simulink library "tip_assist_lib_support"  (Simulink 9.0)
settings: Solver=VariableStepAuto  StartTime=0.0  StopTime=10.0  RelTol=1e-3
undefined symbols (not defined in the file): g, timestep, TipAssistAdvEcmError_t, TipAssistCpmTipOffMode_t, TipAssistLiveWeighStatus_t, TipAssistPayloadType_t, TipAssistSecPfwStatus_t, TipAssistUnsecPfwStatus_t, toa_appNumber, toa_expectedBucketAngNoise, toa_imu_lpf_cutoff_hz, toa_imuBasicOrient, toa_liftBoreDia, toa_liftRodDia, toa_liveLpfCutoffHz, toa_liveSpillRateLpfCutoffHz, toa_mcGroundCombBucketAng, toa_mcGroundCombLiftNormAng, toa_mcGroundLiftNormAng, toa_noSlidingAngle, toa_payload_target_ov_val, toa_payloadTargetMin, toa_pfwLpfCutoffHz, toa_pfwResetLpfCutoffHz, toa_pfwResetStatsBound, toa_pfwResetStatsConf, toa_pfwTiltNormRackThresh, toa_pfwTravelExtentLower, toa_pfwTravelExtentUpper, toa_ratedPayload, toa_reposeMarginAng, toa_sendCpmLiveLpfCutoffHz, toa_sendToCpmMinPrecision, toa_tiltBoreDia, toa_tiltNumCyl, toa_tiltRodDia, toa_toolBcAngle, toa_toolBcLength
libraries: lib_CATutils_Utilities_ApplyName_v2 x113, simulink x18, tip_assist_lib x14, lib_CATutils_Filters_1Pole_LowPass x6, simulink_extras x5, lib_CATutils_Override x3, lib_CATutils_Hysteresis_Latch x3, lib_CATutils_Timer_Countdown x3, tip_assist_lib_support x2
(part 3 of 4)

== system tip_assist_lib_support/Tip-Off Assist Support Lib/Tip-Off Assist Payload/Pseudo-Frictionless Weigh/Notch filter ==
  in : Inport
  reset : Inport  Port=2
  NotchFilter : Subsystem  mask{mskCutoffFreqRadPerSec=5.0}
      mask prompts: mskCutoffFreqRadPerSec "Cutoff Frequency (rad/s)"
      settings: AttributesFormatString=cf: %<mskCutoffFreqRadPerSec>
  NotchFilter1 : Subsystem  mask{mskCutoffFreqRadPerSec=7.5}
      mask prompts: mskCutoffFreqRadPerSec "Cutoff Frequency (rad/s)"
      settings: AttributesFormatString=cf: %<mskCutoffFreqRadPerSec>
  NotchFilter2 : Subsystem  mask{mskCutoffFreqRadPerSec=12.0}
      mask prompts: mskCutoffFreqRadPerSec "Cutoff Frequency (rad/s)"
      settings: AttributesFormatString=cf: %<mskCutoffFreqRadPerSec>
  out : Outport
  wires:
  NotchFilter/1(filtered) -> NotchFilter1/1(raw)
  NotchFilter1/1(filtered) -> NotchFilter2/1(raw)
  reset/1 -> NotchFilter2/2(reset), NotchFilter1/2(reset), NotchFilter/2(reset)
  in/1 -> NotchFilter/1(raw)
  NotchFilter2/1(filtered) -> out/1

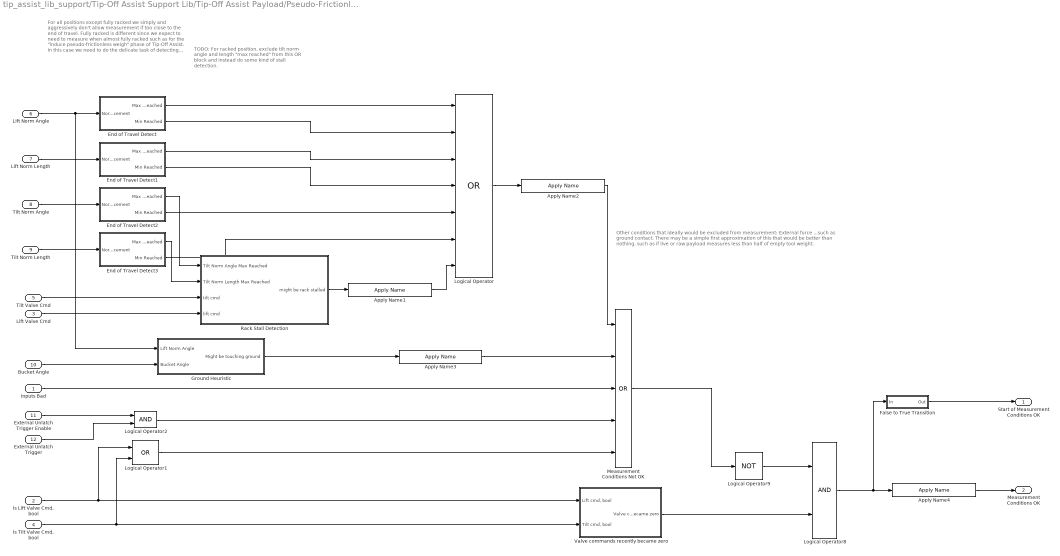
== system tip_assist_lib_support/Tip-Off Assist Support Lib/Tip-Off Assist Payload/Pseudo-Frictionless Weigh/Pseudo-Frictionless Weigh Common Measurement Conditions ==
  note: Other conditions that ideally would be excluded from measurement:
      |
      | External force
      | ...such as ground contact.  There may be a simple first approximation of this that would be better than nothing, such as if live or raw payload measures less than half of empty tool weight.
  note: TODO: For racked position, exclude tilt norm angle and length "max reached" from this OR block and instead do some kind of stall detection.
  note: For all positions except fully racked we simply and aggressively don't allow measurement if too close to the end of travel.
      |
      | Fully racked is different since we expect to need to measure when almost fully racked such as for the "induce pseudo-frictionless weigh" phase of Tip-Off Assist.  In this case we need to do the delicate task of detecting when we are definitely off the rack stops and not hitting the end of tilt cylinder stroke, even if we are close to either.
  Inputs Bad : Inport
  "Is Lift Valve Cmd, bool" : Inport  Port=2
  Lift Valve Cmd : Inport  Port=3
  "Is Tilt Valve Cmd, bool" : Inport  Port=4
  Tilt Valve Cmd : Inport  Port=5
  "Lift Norm Angle " : Inport  Port=6
  Lift Norm Length : Inport  Port=7
  Tilt Norm Angle : Inport  Port=8
  Tilt Norm Length : Inport  Port=9
  Bucket Angle : Inport  Port=10
  External Unlatch Trigger Enable : Inport  Port=11
  External Unlatch Trigger : Inport  Port=12
  Apply Name1 : lib_CATutils_Utilities_ApplyName_v2/Apply Name  sigLabel='toa_pfwMcMaybeRackStall'  enTst=true
  Apply Name2 : lib_CATutils_Utilities_ApplyName_v2/Apply Name  sigLabel='toa_pfwMcMaybeStalled'  enTst=true
  Apply Name3 : lib_CATutils_Utilities_ApplyName_v2/Apply Name  sigLabel='toa_pfwMcMaybeGrounded'  enTst=true
  Apply Name4 : lib_CATutils_Utilities_ApplyName_v2/Apply Name  sigLabel='toa_pfwMcOk'  enTst=true
  End of Travel Detect : Subsystem
  End of Travel Detect1 : Subsystem
  End of Travel Detect2 : Subsystem
  End of Travel Detect3 : Subsystem
  False to True Transition : Subsystem
  Ground Heuristic : Subsystem
  Logical Operator : Logic  Operator=OR  Inputs=7  AllPortsSameDT=off  OutDataTypeStr=boolean
  Logical Operator2 : Logic  AllPortsSameDT=off  OutDataTypeStr=boolean
  Logical Operator1 : Logic  Operator=OR
  Logical Operator8 : Logic
  Logical Operator9 : Logic  Operator=NOT
  Measurement Conditions Not OK : Logic  Operator=OR  Inputs=5  AllPortsSameDT=off  OutDataTypeStr=boolean
  Rack Stall Detection : Subsystem
  Valve commands recently became zero : Subsystem
  Start of Measurement Conditions OK : Outport
  Measurement Conditions OK : Outport  Port=2
  wires:
  False to True Transition/1(Out) -> Start of Measurement Conditions OK/1
  Logical Operator8/1 -> Apply Name4/1, False to True Transition/1(In)
  Inputs Bad/1 -> Measurement Conditions Not OK/3
  Logical Operator9/1 -> Logical Operator8/1
  "Is Lift Valve Cmd, bool"/1 -> Logical Operator1/1, Valve commands recently became zero/1("Lift cmd, bool")
  "Is Tilt Valve Cmd, bool"/1 -> Logical Operator1/2, Valve commands recently became zero/2("Tilt cmd, bool")
  Valve commands recently became zero/1(Valve cmd recently became zero) -> Logical Operator8/2
  Logical Operator/1 -> Apply Name2/1
  Logical Operator1/1 -> Measurement Conditions Not OK/5
  Measurement Conditions Not OK/1 -> Logical Operator9/1
  "Lift Norm Angle "/1 -> Ground Heuristic/1(Lift Norm Angle), End of Travel Detect/1(Normalized Displacement)
  Lift Norm Length/1 -> End of Travel Detect1/1(Normalized Displacement)
  Tilt Norm Angle/1 -> End of Travel Detect2/1(Normalized Displacement)
  End of Travel Detect/2(Min Reached) -> Logical Operator/2
  End of Travel Detect/1(Max Reached) -> Logical Operator/1
  End of Travel Detect1/2(Min Reached) -> Logical Operator/4
  End of Travel Detect1/1(Max Reached) -> Logical Operator/3
  End of Travel Detect2/2(Min Reached) -> Logical Operator/5
  Tilt Norm Length/1 -> End of Travel Detect3/1(Normalized Displacement)
  End of Travel Detect3/2(Min Reached) -> Logical Operator/6
  External Unlatch Trigger/1 -> Logical Operator2/2
  External Unlatch Trigger Enable/1 -> Logical Operator2/1
  Logical Operator2/1 -> Measurement Conditions Not OK/4
  Bucket Angle/1 -> Ground Heuristic/2(Bucket Angle)
  Ground Heuristic/1(Might be touching ground) -> Apply Name3/1
  End of Travel Detect2/1(Max Reached) -> Rack Stall Detection/1(Tilt Norm Angle Max Reached)
  End of Travel Detect3/1(Max Reached) -> Rack Stall Detection/2(Tilt Norm Length Max Reached)
  Tilt Valve Cmd/1 -> Rack Stall Detection/3(tilt cmd)
  Lift Valve Cmd/1 -> Rack Stall Detection/4(lift cmd)
  Rack Stall Detection/1(might be rack stalled) -> Apply Name1/1
  Apply Name4/1 -> Measurement Conditions OK/1
  Apply Name1/1 -> Logical Operator/7
  Apply Name2/1 -> Measurement Conditions Not OK/1
  Apply Name3/1 -> Measurement Conditions Not OK/2

== system tip_assist_lib_support/Tip-Off Assist Support Lib/Tip-Off Assist Payload/Pseudo-Frictionless Weigh/Racked ==
  note: Racking maxes out norm angle or length depending on on lift position. So if one of those is close to 1 we will assume we're racked.
  Tilt Norm Angle : Inport
  Tilt Norm Length : Inport  Port=2
  Add1 : Sum  Inputs=-+
  Data Type Conversion : DataTypeConversion  OutDataTypeStr=boolean
  Latched Point Hysteresis : lib_CATutils_Hysteresis_Latch/Latched Point Hysteresis  extBreakPoints=on  Min_Break_Point=-0.5  Max_Break_Point=0.5  extValues=off  Lo_Value=0  Hi_Value=1  Out_Mode=unused and invalid  Out_DataType=[]  Out_Scaling=[]  OutDataTypeStr=int8
  MinMax : MinMax  Function=max  Inputs=2
  "expected bucket angle noise amplitude, deg" : Constant  Value=toa_expectedBucketAngNoise  OutDataTypeStr=single  SampleTime=-1
  guessed typical ratio of tilt norm angle to bucket angle : Gain  Gain=0.0075
  min tilt norm angle to be considered racked : Constant  Value=toa_pfwTiltNormRackThresh  OutDataTypeStr=single  SampleTime=-1
  "Assume racked, bool" : Outport
  wires:
  Tilt Norm Angle/1 -> MinMax/1
  Data Type Conversion/1 -> "Assume racked, bool"/1
  "expected bucket angle noise amplitude, deg"/1 -> guessed typical ratio of tilt norm angle to bucket angle/1
  Add1/1 -> Latched Point Hysteresis/2
  Latched Point Hysteresis/1 -> Data Type Conversion/1
  min tilt norm angle to be considered racked/1 -> Add1/2, Latched Point Hysteresis/3
  guessed typical ratio of tilt norm angle to bucket angle/1 -> Add1/1
  Tilt Norm Length/1 -> MinMax/2
  MinMax/1 -> Latched Point Hysteresis/1

== system tip_assist_lib_support/Tip-Off Assist Support Lib/Tip-Off Assist Payload/Pseudo-Frictionless Weigh/Secure Latched Payload (resets to NaN) ==
  set : Inport
  reset : Inport  Port=2
  signal : Inport  Port=3
  Unit Delay : UnitDelay  InitialCondition=mskInitialOut  SampleTime=-1
      settings: AttributesFormatString=IC: %<X0>
  false : Constant  Value=mskInitialOut  OutDataTypeStr=Inherit: Inherit via back propagation  SampleTime=-1
  resetSwitch : Switch  Criteria=u2 ~= 0  InputSameDT=on
      settings: AttributesFormatString=%<Criteria>
  setSwitch : Switch  Criteria=u2 ~= 0  InputSameDT=on
      settings: AttributesFormatString=%<Criteria>
  out : Outport
  wires:
  reset/1 -> resetSwitch/2
  setSwitch/1 -> resetSwitch/3
  set/1 -> setSwitch/2
  false/1 -> resetSwitch/1
  signal/1 -> setSwitch/1
  resetSwitch/1 -> out/1, Unit Delay/1
  Unit Delay/1 -> setSwitch/3

== system tip_assist_lib_support/Tip-Off Assist Support Lib/Tip-Off Assist Payload/Pseudo-Frictionless Weigh/Secure Latched Standard Deviation (resets to inf) ==
  set : Inport
  reset : Inport  Port=2
  signal : Inport  Port=3
  Unit Delay : UnitDelay  InitialCondition=mskInitialOut  SampleTime=-1
      settings: AttributesFormatString=IC: %<X0>
  false : Constant  Value=mskInitialOut  OutDataTypeStr=Inherit: Inherit via back propagation  SampleTime=-1
  resetSwitch : Switch  Criteria=u2 ~= 0  InputSameDT=on
      settings: AttributesFormatString=%<Criteria>
  setSwitch : Switch  Criteria=u2 ~= 0  InputSameDT=on
      settings: AttributesFormatString=%<Criteria>
  out : Outport
  wires:
  Unit Delay/1 -> setSwitch/3
  resetSwitch/1 -> Unit Delay/1, out/1
  signal/1 -> setSwitch/1
  false/1 -> resetSwitch/1
  set/1 -> setSwitch/2
  setSwitch/1 -> resetSwitch/3
  reset/1 -> resetSwitch/2

== system tip_assist_lib_support/Tip-Off Assist Support Lib/Tip-Off Assist Payload/Pseudo-Frictionless Weigh/Secure Payload Latch State ==
  set : Inport
  reset : Inport  Port=2
  Unit Delay : UnitDelay  InitialCondition=mskInitialOut  SampleTime=-1
      settings: AttributesFormatString=IC: %<X0>
  false : Constant  Value=0  OutDataTypeStr=boolean
  resetSwitch : Switch  Criteria=u2 ~= 0  InputSameDT=on
      settings: AttributesFormatString=%<Criteria>
  setSwitch : Switch  Criteria=u2 ~= 0  InputSameDT=on
      settings: AttributesFormatString=%<Criteria>
  true : Constant  OutDataTypeStr=boolean
  out : Outport
  wires:
  Unit Delay/1 -> setSwitch/3
  resetSwitch/1 -> Unit Delay/1, out/1
  true/1 -> setSwitch/1
  false/1 -> resetSwitch/1
  set/1 -> setSwitch/2
  setSwitch/1 -> resetSwitch/3
  reset/1 -> resetSwitch/2

== system tip_assist_lib_support/Tip-Off Assist Support Lib/Tip-Off Assist Payload/Pseudo-Frictionless Weigh/Secure Payload Unlatch Logic ==
  note: When external unlatch is disabled, the non-command unlatch signals become relevant if slope is used. The noise in the slope would need to be accounted for somewhere to prevent accidental unlatching.
  Lift Cmd : Inport
  Tilt Cmd : Inport  Port=2
  External Unlatch Trigger Enable : Inport  Port=3
  External Unlatch Trigger : Inport  Port=4
  Unsecure Transition Unlatch Trigger : Inport  Port=5
  Apply Name1 : lib_CATutils_Utilities_ApplyName_v2/Apply Name  sigLabel='toa_pfwLatchInvalidate'  enTst=true
  Logical Operator2 : Logic  Operator=OR  AllPortsSameDT=off  OutDataTypeStr=boolean
  Logical Operator3 : Logic  Operator=OR  AllPortsSameDT=off  OutDataTypeStr=boolean
  Switch : Switch  Criteria=u2 ~= 0
  Unlatch Out : Outport
  wires:
  Switch/1 -> Apply Name1/1
  External Unlatch Trigger/1 -> Logical Operator3/1
  External Unlatch Trigger Enable/1 -> Switch/2
  Lift Cmd/1 -> Logical Operator2/1
  Tilt Cmd/1 -> Logical Operator2/2
  Logical Operator2/1 -> Switch/3
  Unsecure Transition Unlatch Trigger/1 -> Logical Operator3/2
  Logical Operator3/1 -> Switch/1
  Apply Name1/1 -> Unlatch Out/1

== system tip_assist_lib_support/Tip-Off Assist Support Lib/Tip-Off Assist Payload/Pseudo-Frictionless Weigh/Sliding ==
  "Bucket Angle, deg" : Inport
  Add1 : Sum
  Data Type Conversion : DataTypeConversion  OutDataTypeStr=boolean
  Latched Point Hysteresis : lib_CATutils_Hysteresis_Latch/Latched Point Hysteresis  extBreakPoints=on  Min_Break_Point=-0.5  Max_Break_Point=0.5  extValues=off  Lo_Value=0  Hi_Value=1  Out_Mode=unused and invalid  Out_DataType=[]  Out_Scaling=[]  OutDataTypeStr=int8
  "expected bucket angle noise amplitude, deg" : Constant  Value=toa_expectedBucketAngNoise  OutDataTypeStr=single  SampleTime=-1
  "sliding threshold, degrees" : Constant  Value=toa_noSlidingAngle  OutDataTypeStr=single  SampleTime=-1
  "Assume no sliding, bool" : Outport
  "Bucket angle of no sliding threshold, deg" : Outport  Port=2
  wires:
  "sliding threshold, degrees"/1 -> "Bucket angle of no sliding threshold, deg"/1, Add1/1, Latched Point Hysteresis/2
  Latched Point Hysteresis/1 -> Data Type Conversion/1
  Add1/1 -> Latched Point Hysteresis/3
  "expected bucket angle noise amplitude, deg"/1 -> Add1/2
  Data Type Conversion/1 -> "Assume no sliding, bool"/1
  "Bucket Angle, deg"/1 -> Latched Point Hysteresis/1

== system tip_assist_lib_support/Tip-Off Assist Support Lib/Tip-Off Assist Payload/Pseudo-Frictionless Weigh/Statistics Estimation1 ==
  note: A good variance to reset the filter to is the variance that corresponds to the distribution whose confidence interval at the prescribed confidence (99.7%) has a half-width (aka bound) that is 75% of the rated payload.
      |
      | This is like saying that we're always 99.7% sure that the true payload is within 75% of rated payload of our raw measurement.
  Signal In : Inport
  Low Pass Filter Cutoff (Hz) : Inport  Port=2
  Reset : Inport  Port=3
  "Rated Payload, t" : Inport  Port=4
  Constant : Constant  Value=toa_pfwResetStatsConf  OutDataTypeStr=single  SampleTime=-1
  Constant1 : Constant  Value=toa_pfwResetStatsBound  OutDataTypeStr=single  SampleTime=-1
  Constant2 : Constant  Value=timestep  SampleTime=timestep
  MATLAB Function : MATLAB Function  TreatAsAtomicUnit=on
  MATLAB Function1 : tip_assist_lib/MATLAB Function
  Math Function : Math  Operator=square  SaturateOnIntegerOverflow=on
  Product : Product
  Two Sided St. Dev. from Bound : MATLAB Function  TreatAsAtomicUnit=on
  stdevEst : Outport
  meanEst : Outport  Port=2
  wires:
  Reset/1 -> MATLAB Function/3(reset)
  MATLAB Function1/1 -> MATLAB Function/2(filterFactor)
  Low Pass Filter Cutoff (Hz)/1 -> MATLAB Function1/2
  Constant2/1 -> MATLAB Function1/1
  MATLAB Function/2(stdevEst) -> stdevEst/1
  MATLAB Function/1(meanEst) -> meanEst/1
  Signal In/1 -> MATLAB Function/4(resetSample), MATLAB Function/1(newSample)
  "Rated Payload, t"/1 -> Product/1
  Constant/1 -> Two Sided St. Dev. from Bound/1(confidence)
  Math Function/1 -> MATLAB Function/5(resetVariance)
  Two Sided St. Dev. from Bound/1(stdev) -> Math Function/1
  Constant1/1 -> Product/2
  Product/1 -> Two Sided St. Dev. from Bound/2(bound)

== system tip_assist_lib_support/Tip-Off Assist Support Lib/Tip-Off Assist Payload/Pseudo-Frictionless Weigh/Statistics Estimation2 ==
  note: A good variance to reset the filter to is the variance that corresponds to the distribution whose confidence interval at the prescribed confidence (99.7%) has a half-width (aka bound) that is 75% of the rated payload.
      |
      | This is like saying that we're always 99.7% sure that the true payload is within 75% of rated payload of our raw measurement.
  Signal In : Inport
  Low Pass Filter Cutoff (Hz) : Inport  Port=2
  Reset : Inport  Port=3
  "Rated Payload, t" : Inport  Port=4
  Constant : Constant  Value=toa_pfwResetStatsConf  OutDataTypeStr=single  SampleTime=-1
  Constant1 : Constant  Value=toa_pfwResetStatsBound  OutDataTypeStr=single  SampleTime=-1
  Constant2 : Constant  Value=timestep  SampleTime=timestep
  MATLAB Function : MATLAB Function  TreatAsAtomicUnit=on
  MATLAB Function1 : tip_assist_lib/MATLAB Function
  Math Function : Math  Operator=square  SaturateOnIntegerOverflow=on
  Product : Product
  Two Sided St. Dev. from Bound : MATLAB Function  TreatAsAtomicUnit=on
  stdevEst : Outport
  meanEst : Outport  Port=2
  wires:
  Product/1 -> Two Sided St. Dev. from Bound/2(bound)
  Constant1/1 -> Product/2
  Two Sided St. Dev. from Bound/1(stdev) -> Math Function/1
  Math Function/1 -> MATLAB Function/5(resetVariance)
  Constant/1 -> Two Sided St. Dev. from Bound/1(confidence)
  "Rated Payload, t"/1 -> Product/1
  Signal In/1 -> MATLAB Function/4(resetSample), MATLAB Function/1(newSample)
  MATLAB Function/1(meanEst) -> meanEst/1
  MATLAB Function/2(stdevEst) -> stdevEst/1
  Constant2/1 -> MATLAB Function1/1
  Low Pass Filter Cutoff (Hz)/1 -> MATLAB Function1/2
  MATLAB Function1/1 -> MATLAB Function/2(filterFactor)
  Reset/1 -> MATLAB Function/3(reset)

== system tip_assist_lib_support/Tip-Off Assist Support Lib/Tip-Off Assist Payload/Pseudo-Frictionless Weigh/Sure dig is over ==
  note: need a set/reset block here so we can only call a dig over if we previously knew a dig was happening
  note: need a timer here so that if dig starts but we never see anything saying its over we call it over a certain amount of time after dig state becomes false
  note: need a block here that looks for a definite dump
  Dig State : Inport
  Ground Speed : Inport  Port=2
  Ground Speed1 : Inport  Port=3
  Tilt Cmd : Inport  Port=4
  Logical Operator : Logic  Operator=OR  AllPortsSameDT=off  OutDataTypeStr=boolean
  Dig Definitely Done event : Outport
  wires:
  Dig State/1 -> ?
  Logical Operator/1 -> Dig Definitely Done event/1

== system tip_assist_lib_support/Tip-Off Assist Support Lib/Tip-Off Assist Payload/Pseudo-Frictionless Weigh/Variance Anti-Noise Filter1 ==
  note: Per Aaron Shatters:
      | This filter was added to PCS (the CPM predecessor) because pump piston pass frequency was aliasing into the signal.  Being kind of like a discrete derivative, the variance calculation is sensitive to high frequency noise.  So this filter was added to prevent the high frequency instances of this noise.  Being a two sample moving average, it is the fastest filter that eliminated the noise.  It was not thoroughly technically examined, but it worked.  It's not clear the extent to which this is necessary here, since Pseudo-Frictionless Weigh works only when the tilt and lift valve command is zero, so the pump should not be hydraulically connected to the cylinder at this time.  The pump is also likely to be at a low stroke, so piston pass ripple amplitude should be low.
  in : Inport
  reset : Inport  Port=2
  MATLAB Function : MATLAB Function  TreatAsAtomicUnit=on
  out : Outport
  wires:
  reset/1 -> MATLAB Function/2(reset)
  in/1 -> MATLAB Function/1(u)
  MATLAB Function/1(y) -> out/1

== system tip_assist_lib_support/Tip-Off Assist Support Lib/Tip-Off Assist Payload/Pseudo-Frictionless Weigh/Variance Anti-Noise Filter2 ==
  note: Per Aaron Shatters:
      | This filter was added to PCS (the CPM predecessor) because pump piston pass frequency was aliasing into the signal.  Being kind of like a discrete derivative, the variance calculation is sensitive to high frequency noise.  So this filter was added to prevent the high frequency instances of this noise.  Being a two sample moving average, it is the fastest filter that eliminated the noise.  It was not thoroughly technically examined, but it worked.  It's not clear the extent to which this is necessary here, since Pseudo-Frictionless Weigh works only when the tilt and lift valve command is zero, so the pump should not be hydraulically connected to the cylinder at this time.  The pump is also likely to be at a low stroke, so piston pass ripple amplitude should be low.
  in : Inport
  reset : Inport  Port=2
  MATLAB Function : MATLAB Function  TreatAsAtomicUnit=on
  out : Outport
  wires:
  MATLAB Function/1(y) -> out/1
  in/1 -> MATLAB Function/1(u)
  reset/1 -> MATLAB Function/2(reset)

== system tip_assist_lib_support/Tip-Off Assist Support Lib/Tip-Off Assist Payload/Pseudo-Frictionless Weigh/Weighing Statistics, No Notch, No Latch ==
  PFW Payload Std. Dev. : Inport
  PFW Payload Mean : Inport  Port=2
  Add : Sum
  Add1 : Sum
  Constant : Constant  Value=0.997
  One Sided Confidence Limit : MATLAB Function  TreatAsAtomicUnit=on
  Subtract : Sum  Inputs=+-
  Subtract1 : Sum  Inputs=+-
  Two Sided Confidence Limit : MATLAB Function  TreatAsAtomicUnit=on
  One Sided Payload Upper Bound : Outport
  One Sided Payload Lower Bound : Outport  Port=2
  One Sided Payload Bound Size : Outport  Port=3
  Two Sided Payload Upper Bound : Outport  Port=4
  Two Sided Payload Lower Bound : Outport  Port=5
  Two Sided Payload Bound Size : Outport  Port=6
  wires:
  PFW Payload Mean/1 -> Subtract1/1, Add1/2, Subtract/1, Add/2
  PFW Payload Std. Dev./1 -> Two Sided Confidence Limit/2(stdev), One Sided Confidence Limit/2(stdev)
  Constant/1 -> One Sided Confidence Limit/1(confidence), Two Sided Confidence Limit/1(confidence)
  One Sided Confidence Limit/1(bound) -> Subtract/2, Add/1, One Sided Payload Bound Size/1
  Add/1 -> One Sided Payload Upper Bound/1
  Subtract/1 -> One Sided Payload Lower Bound/1
  Two Sided Confidence Limit/1(bound) -> Subtract1/2, Add1/1, Two Sided Payload Bound Size/1
  Add1/1 -> Two Sided Payload Upper Bound/1
  Subtract1/1 -> Two Sided Payload Lower Bound/1

== system tip_assist_lib_support/Tip-Off Assist Support Lib/Tip-Off Assist Payload/Pseudo-Frictionless Weigh/Weighing Statistics, Notch, No Latch ==
  PFW Payload Std. Dev. : Inport
  PFW Payload Mean : Inport  Port=2
  Add : Sum
  Add1 : Sum
  Constant : Constant  Value=0.997
  One Sided Confidence Limit : MATLAB Function  TreatAsAtomicUnit=on
  Subtract : Sum  Inputs=+-
  Subtract1 : Sum  Inputs=+-
  Two Sided Confidence Limit : MATLAB Function  TreatAsAtomicUnit=on
  One Sided Payload Upper Bound : Outport
  One Sided Payload Lower Bound : Outport  Port=2
  One Sided Payload Bound Size : Outport  Port=3
  Two Sided Payload Upper Bound : Outport  Port=4
  Two Sided Payload Lower Bound : Outport  Port=5
  Two Sided Payload Bound Size : Outport  Port=6
  wires:
  Subtract1/1 -> Two Sided Payload Lower Bound/1
  Add1/1 -> Two Sided Payload Upper Bound/1
  Two Sided Confidence Limit/1(bound) -> Two Sided Payload Bound Size/1, Add1/1, Subtract1/2
  Subtract/1 -> One Sided Payload Lower Bound/1
  Add/1 -> One Sided Payload Upper Bound/1
  One Sided Confidence Limit/1(bound) -> One Sided Payload Bound Size/1, Add/1, Subtract/2
  Constant/1 -> Two Sided Confidence Limit/1(confidence), One Sided Confidence Limit/1(confidence)
  PFW Payload Std. Dev./1 -> One Sided Confidence Limit/2(stdev), Two Sided Confidence Limit/2(stdev)
  PFW Payload Mean/1 -> Add/2, Subtract/1, Add1/2, Subtract1/1

== system tip_assist_lib_support/Tip-Off Assist Support Lib/Tip-Off Assist Payload/Pseudo-Frictionless Weigh/Weighing Statistics, Secure Latched ==
  PFW Payload Std. Dev. : Inport
  PFW Payload Mean : Inport  Port=2
  Add : Sum
  Add1 : Sum
  Constant : Constant  Value=0.997
  One Sided Confidence Limit : MATLAB Function  TreatAsAtomicUnit=on
  Subtract : Sum  Inputs=+-
  Subtract1 : Sum  Inputs=+-
  Two Sided Confidence Limit : MATLAB Function  TreatAsAtomicUnit=on
  One Sided Payload Upper Bound : Outport
  One Sided Payload Lower Bound : Outport  Port=2
  One Sided Payload Bound Size : Outport  Port=3
  Two Sided Payload Upper Bound : Outport  Port=4
  Two Sided Payload Lower Bound : Outport  Port=5
  Two Sided Payload Bound Size : Outport  Port=6
  wires:
  PFW Payload Mean/1 -> Subtract1/1, Add1/2, Subtract/1, Add/2
  PFW Payload Std. Dev./1 -> Two Sided Confidence Limit/2(stdev), One Sided Confidence Limit/2(stdev)
  Constant/1 -> One Sided Confidence Limit/1(confidence), Two Sided Confidence Limit/1(confidence)
  One Sided Confidence Limit/1(bound) -> One Sided Payload Bound Size/1, Subtract/2, Add/1
  Add/1 -> One Sided Payload Upper Bound/1
  Subtract/1 -> One Sided Payload Lower Bound/1
  Two Sided Confidence Limit/1(bound) -> Two Sided Payload Bound Size/1, Subtract1/2, Add1/1
  Add1/1 -> Two Sided Payload Upper Bound/1
  Subtract1/1 -> Two Sided Payload Lower Bound/1

== system tip_assist_lib_support/Tip-Off Assist Support Lib/Tip-Off Assist Payload/Live Weigh/Notch filter/NotchFilter ==
  raw : Inport
  reset : Inport  Port=2
  Constant : Constant  Value=mskCutoffFreqRadPerSec  OutDataTypeStr=Inherit: Inherit via back propagation
  Data Type Duplicate : DataTypeDuplicate
  Data Type Conversion : DataTypeConversion
  Data Type Conversion1 : DataTypeConversion  SaturateOnIntegerOverflow=on
  Filter : Stateflow chart  TreatAsAtomicUnit=on
  Weighted Sample Time : SampleTimeMath  TsampMathOp=Ts Only  OutDataTypeStr=Inherit: Inherit via back propagation
  filtered : Outport
  wires:
  Filter/1(filtered) -> Data Type Conversion1/1
  reset/1 -> Filter/2(reset)
  Weighted Sample Time/1 -> Filter/3(ts)
  Constant/1 -> Filter/4(cf)
  Data Type Conversion/1 -> Filter/1(raw)
  Data Type Conversion1/1 -> Data Type Duplicate/2, filtered/1
  raw/1 -> Weighted Sample Time/1, Data Type Duplicate/1, Data Type Conversion/1

== system tip_assist_lib_support/Tip-Off Assist Support Lib/Tip-Off Assist Payload/Live Weigh/Notch filter/NotchFilter1 ==
  raw : Inport
  reset : Inport  Port=2
  Constant : Constant  Value=mskCutoffFreqRadPerSec  OutDataTypeStr=Inherit: Inherit via back propagation
  Data Type Duplicate : DataTypeDuplicate
  Data Type Conversion : DataTypeConversion
  Data Type Conversion1 : DataTypeConversion  SaturateOnIntegerOverflow=on
  Filter : Stateflow chart  TreatAsAtomicUnit=on
  Weighted Sample Time : SampleTimeMath  TsampMathOp=Ts Only  OutDataTypeStr=Inherit: Inherit via back propagation
  filtered : Outport
  wires:
  Filter/1(filtered) -> Data Type Conversion1/1
  reset/1 -> Filter/2(reset)
  Weighted Sample Time/1 -> Filter/3(ts)
  Constant/1 -> Filter/4(cf)
  Data Type Conversion/1 -> Filter/1(raw)
  Data Type Conversion1/1 -> Data Type Duplicate/2, filtered/1
  raw/1 -> Weighted Sample Time/1, Data Type Duplicate/1, Data Type Conversion/1

== system tip_assist_lib_support/Tip-Off Assist Support Lib/Tip-Off Assist Payload/Live Weigh/Notch filter/NotchFilter2 ==
  raw : Inport
  reset : Inport  Port=2
  Constant : Constant  Value=mskCutoffFreqRadPerSec  OutDataTypeStr=Inherit: Inherit via back propagation
  Data Type Duplicate : DataTypeDuplicate
  Data Type Conversion : DataTypeConversion
  Data Type Conversion1 : DataTypeConversion  SaturateOnIntegerOverflow=on
  Filter : Stateflow chart  TreatAsAtomicUnit=on
  Weighted Sample Time : SampleTimeMath  TsampMathOp=Ts Only  OutDataTypeStr=Inherit: Inherit via back propagation
  filtered : Outport
  wires:
  Filter/1(filtered) -> Data Type Conversion1/1
  reset/1 -> Filter/2(reset)
  Weighted Sample Time/1 -> Filter/3(ts)
  Constant/1 -> Filter/4(cf)
  Data Type Conversion/1 -> Filter/1(raw)
  Data Type Conversion1/1 -> Data Type Duplicate/2, filtered/1
  raw/1 -> Weighted Sample Time/1, Data Type Duplicate/1, Data Type Conversion/1

== system tip_assist_lib_support/Tip-Off Assist Support Lib/Tip-Off Assist Payload/Pseudo-Frictionless Weigh/Collapsing/Minimum Angle For Current Load (resets to 99) ==
  set : Inport
  reset : Inport  Port=2
  signal : Inport  Port=3
  Unit Delay : UnitDelay  InitialCondition=mskInitialOut  SampleTime=-1
      settings: AttributesFormatString=IC: %<X0>
  false : Constant  Value=mskInitialOut  OutDataTypeStr=Inherit: Inherit via back propagation  SampleTime=-1
  resetSwitch : Switch  Criteria=u2 ~= 0  InputSameDT=on
      settings: AttributesFormatString=%<Criteria>
  setSwitch : Switch  Criteria=u2 ~= 0  InputSameDT=on
      settings: AttributesFormatString=%<Criteria>
  out : Outport
  wires:
  reset/1 -> resetSwitch/2
  setSwitch/1 -> resetSwitch/3
  set/1 -> setSwitch/2
  false/1 -> resetSwitch/1
  signal/1 -> setSwitch/1
  resetSwitch/1 -> out/1, Unit Delay/1
  Unit Delay/1 -> setSwitch/3

== system tip_assist_lib_support/Tip-Off Assist Support Lib/Tip-Off Assist Payload/Pseudo-Frictionless Weigh/Notch filter/NotchFilter ==
  raw : Inport
  reset : Inport  Port=2
  Constant : Constant  Value=mskCutoffFreqRadPerSec  OutDataTypeStr=Inherit: Inherit via back propagation
  Data Type Duplicate : DataTypeDuplicate
  Data Type Conversion : DataTypeConversion
  Data Type Conversion1 : DataTypeConversion  SaturateOnIntegerOverflow=on
  Filter : Stateflow chart  TreatAsAtomicUnit=on
  Weighted Sample Time : SampleTimeMath  TsampMathOp=Ts Only  OutDataTypeStr=Inherit: Inherit via back propagation
  filtered : Outport
  wires:
  Filter/1(filtered) -> Data Type Conversion1/1
  reset/1 -> Filter/2(reset)
  Weighted Sample Time/1 -> Filter/3(ts)
  Constant/1 -> Filter/4(cf)
  Data Type Conversion/1 -> Filter/1(raw)
  Data Type Conversion1/1 -> Data Type Duplicate/2, filtered/1
  raw/1 -> Weighted Sample Time/1, Data Type Duplicate/1, Data Type Conversion/1

== system tip_assist_lib_support/Tip-Off Assist Support Lib/Tip-Off Assist Payload/Pseudo-Frictionless Weigh/Notch filter/NotchFilter1 ==
  raw : Inport
  reset : Inport  Port=2
  Constant : Constant  Value=mskCutoffFreqRadPerSec  OutDataTypeStr=Inherit: Inherit via back propagation
  Data Type Duplicate : DataTypeDuplicate
  Data Type Conversion : DataTypeConversion
  Data Type Conversion1 : DataTypeConversion  SaturateOnIntegerOverflow=on
  Filter : Stateflow chart  TreatAsAtomicUnit=on
  Weighted Sample Time : SampleTimeMath  TsampMathOp=Ts Only  OutDataTypeStr=Inherit: Inherit via back propagation
  filtered : Outport
  wires:
  Filter/1(filtered) -> Data Type Conversion1/1
  reset/1 -> Filter/2(reset)
  Weighted Sample Time/1 -> Filter/3(ts)
  Constant/1 -> Filter/4(cf)
  Data Type Conversion/1 -> Filter/1(raw)
  Data Type Conversion1/1 -> Data Type Duplicate/2, filtered/1
  raw/1 -> Weighted Sample Time/1, Data Type Duplicate/1, Data Type Conversion/1

== system tip_assist_lib_support/Tip-Off Assist Support Lib/Tip-Off Assist Payload/Pseudo-Frictionless Weigh/Notch filter/NotchFilter2 ==
  raw : Inport
  reset : Inport  Port=2
  Constant : Constant  Value=mskCutoffFreqRadPerSec  OutDataTypeStr=Inherit: Inherit via back propagation
  Data Type Duplicate : DataTypeDuplicate
  Data Type Conversion : DataTypeConversion
  Data Type Conversion1 : DataTypeConversion  SaturateOnIntegerOverflow=on
  Filter : Stateflow chart  TreatAsAtomicUnit=on
  Weighted Sample Time : SampleTimeMath  TsampMathOp=Ts Only  OutDataTypeStr=Inherit: Inherit via back propagation
  filtered : Outport
  wires:
  Filter/1(filtered) -> Data Type Conversion1/1
  reset/1 -> Filter/2(reset)
  Weighted Sample Time/1 -> Filter/3(ts)
  Constant/1 -> Filter/4(cf)
  Data Type Conversion/1 -> Filter/1(raw)
  Data Type Conversion1/1 -> Data Type Duplicate/2, filtered/1
  raw/1 -> Weighted Sample Time/1, Data Type Duplicate/1, Data Type Conversion/1

== system tip_assist_lib_support/Tip-Off Assist Support Lib/Tip-Off Assist Payload/Pseudo-Frictionless Weigh/Pseudo-Frictionless Weigh Common Measurement Conditions/End of Travel Detect ==
  Normalized Displacement : Inport
  Max travel : Constant  Value=toa_pfwTravelExtentUpper  OutDataTypeStr=single  SampleTime=-1
  Min travel : Constant  Value=toa_pfwTravelExtentLower  OutDataTypeStr=single  SampleTime=-1
  Relational Operator : RelationalOperator  RndMeth=Nearest  InputSameDT=on
  Relational Operator1 : RelationalOperator  Operator=<=  RndMeth=Nearest  InputSameDT=on
  Max Reached : Outport
  Min Reached : Outport  Port=2
  wires:
  Normalized Displacement/1 -> Relational Operator1/1, Relational Operator/1
  Max travel/1 -> Relational Operator/2
  Min travel/1 -> Relational Operator1/2
  Relational Operator/1 -> Max Reached/1
  Relational Operator1/1 -> Min Reached/1

== system tip_assist_lib_support/Tip-Off Assist Support Lib/Tip-Off Assist Payload/Pseudo-Frictionless Weigh/Pseudo-Frictionless Weigh Common Measurement Conditions/End of Travel Detect1 ==
  Normalized Displacement : Inport
  Max travel : Constant  Value=toa_pfwTravelExtentUpper  OutDataTypeStr=single  SampleTime=-1
  Min travel : Constant  Value=toa_pfwTravelExtentLower  OutDataTypeStr=single  SampleTime=-1
  Relational Operator : RelationalOperator  RndMeth=Nearest  InputSameDT=on
  Relational Operator1 : RelationalOperator  Operator=<=  RndMeth=Nearest  InputSameDT=on
  Max Reached : Outport
  Min Reached : Outport  Port=2
  wires:
  Relational Operator1/1 -> Min Reached/1
  Relational Operator/1 -> Max Reached/1
  Min travel/1 -> Relational Operator1/2
  Max travel/1 -> Relational Operator/2
  Normalized Displacement/1 -> Relational Operator/1, Relational Operator1/1

== system tip_assist_lib_support/Tip-Off Assist Support Lib/Tip-Off Assist Payload/Pseudo-Frictionless Weigh/Pseudo-Frictionless Weigh Common Measurement Conditions/End of Travel Detect2 ==
  Normalized Displacement : Inport
  Max travel : Constant  Value=toa_pfwTravelExtentUpper  OutDataTypeStr=single  SampleTime=-1
  Min travel : Constant  Value=toa_pfwTravelExtentLower  OutDataTypeStr=single  SampleTime=-1
  Relational Operator : RelationalOperator  RndMeth=Nearest  InputSameDT=on
  Relational Operator1 : RelationalOperator  Operator=<=  RndMeth=Nearest  InputSameDT=on
  Max Reached : Outport
  Min Reached : Outport  Port=2
  wires:
  Relational Operator1/1 -> Min Reached/1
  Relational Operator/1 -> Max Reached/1
  Min travel/1 -> Relational Operator1/2
  Max travel/1 -> Relational Operator/2
  Normalized Displacement/1 -> Relational Operator/1, Relational Operator1/1

== system tip_assist_lib_support/Tip-Off Assist Support Lib/Tip-Off Assist Payload/Pseudo-Frictionless Weigh/Pseudo-Frictionless Weigh Common Measurement Conditions/End of Travel Detect3 ==
  Normalized Displacement : Inport
  Max travel : Constant  Value=toa_pfwTravelExtentUpper  OutDataTypeStr=single  SampleTime=-1
  Min travel : Constant  Value=toa_pfwTravelExtentLower  OutDataTypeStr=single  SampleTime=-1
  Relational Operator : RelationalOperator  RndMeth=Nearest  InputSameDT=on
  Relational Operator1 : RelationalOperator  Operator=<=  RndMeth=Nearest  InputSameDT=on
  Max Reached : Outport
  Min Reached : Outport  Port=2
  wires:
  Relational Operator1/1 -> Min Reached/1
  Relational Operator/1 -> Max Reached/1
  Min travel/1 -> Relational Operator1/2
  Max travel/1 -> Relational Operator/2
  Normalized Displacement/1 -> Relational Operator/1, Relational Operator1/1

== system tip_assist_lib_support/Tip-Off Assist Support Lib/Tip-Off Assist Payload/Pseudo-Frictionless Weigh/Pseudo-Frictionless Weigh Common Measurement Conditions/False to True Transition ==
  In : Inport
  Compare to Constant : simulink/Logic and Bit Operations/Compare To Constant  relop===  const=0  OutDataTypeStr=boolean
      settings: AttributesFormatString=Operator: %<relop>\nConst: %<const>
  Compare to Constant1 : simulink/Logic and Bit Operations/Compare To Constant  relop===  const=1  OutDataTypeStr=boolean
      settings: AttributesFormatString=Operator: %<relop>\nConst: %<const>
  Delay : Delay  DelayLength=1
  Logical Operator : Logic
  Out : Outport
  wires:
  In/1 -> Compare to Constant1/1, Delay/1
  Logical Operator/1 -> Out/1
  Compare to Constant/1 -> Logical Operator/2
  Delay/1 -> Compare to Constant/1
  Compare to Constant1/1 -> Logical Operator/1

== system tip_assist_lib_support/Tip-Off Assist Support Lib/Tip-Off Assist Payload/Pseudo-Frictionless Weigh/Pseudo-Frictionless Weigh Common Measurement Conditions/Ground Heuristic ==
  Lift Norm Angle : Inport
  Bucket Angle : Inport  Port=2
  Constant : Constant  Value=toa_mcGroundCombLiftNormAng  OutDataTypeStr=single  SampleTime=-1
  Constant1 : Constant  Value=toa_mcGroundCombBucketAng  OutDataTypeStr=single  SampleTime=-1
  Constant2 : Constant  Value=toa_mcGroundLiftNormAng  OutDataTypeStr=single  SampleTime=-1
  Logical Operator1 : Logic  Operator=OR  AllPortsSameDT=off  OutDataTypeStr=boolean
  Logical Operator3 : Logic  AllPortsSameDT=off  OutDataTypeStr=boolean
  Relational Operator : RelationalOperator  Operator=<=  OutDataTypeStr=boolean  RndMeth=Simplest
  Relational Operator1 : RelationalOperator  Operator=<=  OutDataTypeStr=boolean  RndMeth=Simplest
  Relational Operator2 : RelationalOperator  Operator=<=  OutDataTypeStr=boolean  RndMeth=Simplest
  Might be touching ground : Outport
  wires:
  Relational Operator1/1 -> Logical Operator3/2
  Logical Operator3/1 -> Logical Operator1/2
  Bucket Angle/1 -> Relational Operator1/1
  Relational Operator/1 -> Logical Operator3/1
  Constant/1 -> Relational Operator/2
  Lift Norm Angle/1 -> Relational Operator2/1, Relational Operator/1
  Constant1/1 -> Relational Operator1/2
  Logical Operator1/1 -> Might be touching ground/1
  Relational Operator2/1 -> Logical Operator1/1
  Constant2/1 -> Relational Operator2/2

== system tip_assist_lib_support/Tip-Off Assist Support Lib/Tip-Off Assist Payload/Pseudo-Frictionless Weigh/Pseudo-Frictionless Weigh Common Measurement Conditions/Rack Stall Detection ==
  note: Dumping proves can't be rack stalled - unless we've lowered, because it is possible to lower into the rack stops.
  Tilt Norm Angle Max Reached : Inport
  Tilt Norm Length Max Reached : Inport  Port=2
  tilt cmd : Inport  Port=3
  lift cmd : Inport  Port=4
  Constant : Constant  Value=true  SampleTime=-1
  Dumping : simulink/Logic and Bit Operations/Compare To Constant  relop=<  const=0  OutDataTypeStr=boolean
  Logical Operator3 : Logic  AllPortsSameDT=off  OutDataTypeStr=boolean
  Logical Operator4 : Logic  Operator=OR  AllPortsSameDT=off  OutDataTypeStr=boolean
  Lowering : simulink/Logic and Bit Operations/Compare To Constant  relop=<  const=0  OutDataTypeStr=boolean
  Might be rack stalled based on position only : Logic  Operator=OR  AllPortsSameDT=off  OutDataTypeStr=boolean
  Racking : simulink/Logic and Bit Operations/Compare To Constant  relop=>  const=0  OutDataTypeStr=boolean
  Valve command history proves not rack stalled (resets to false) : tip_assist_lib_support/Tip-Off Assist Support Lib/Tip-Off Assist Payload/Pseudo-Frictionless Weigh/Collapsing/Minimum Angle For Current Load (resets to 99)  mskInitialOut=false
  not : Logic  Operator=NOT  AllPortsSameDT=off  OutDataTypeStr=boolean
  might be rack stalled : Outport
  wires:
  Valve command history proves not rack stalled (resets to false)/1 -> not/1  "proved not rack stalled"
  Might be rack stalled based on position only/1 -> Logical Operator3/1
  Lowering/1 -> Logical Operator4/2
  Logical Operator3/1 -> might be rack stalled/1  "maybe rack stalled"
  Logical Operator4/1 -> Valve command history proves not rack stalled (resets to false)/2
  Dumping/1 -> Valve command history proves not rack stalled (resets to false)/1
  lift cmd/1 -> Lowering/1
  Constant/1 -> Valve command history proves not rack stalled (resets to false)/3
  not/1 -> Logical Operator3/2  "can't prove not rack stalled"
  Tilt Norm Angle Max Reached/1 -> Might be rack stalled based on position only/1
  Tilt Norm Length Max Reached/1 -> Might be rack stalled based on position only/2
  Racking/1 -> Logical Operator4/1
  tilt cmd/1 -> Racking/1, Dumping/1

== system tip_assist_lib_support/Tip-Off Assist Support Lib/Tip-Off Assist Payload/Pseudo-Frictionless Weigh/Pseudo-Frictionless Weigh Common Measurement Conditions/Valve commands recently became zero ==
  note: Some time after the function is in the hold position, leakage starts to transfer some of the borne weight to static friction between the piston and cylinder bore, which we can't measure. So we only allow measurement for a certain time after the hold position. If one day it becomes desirable to be able to measure for longer, this could be possible by removing the expiration (or making it longer) and introducing some model of leakage to compensate and produce an "effective" pressure instead of actual pressure. Effective pressure would represent the expected static friction force as pressure. CPM already does something like this for the lift cylinders.
  "Lift cmd, bool" : Inport
  "Tilt cmd, bool" : Inport  Port=2
  Lift expired? : lib_CATutils_Timer_Countdown/Timer Countdown  initTime=toa_pfw_time_limit  maxTime=400  timingInput=True  expiredOutput=True  initState=False
  Logical Operator{,3..5} (4 alike) : Logic  Operator=NOT
  Logical Operator1 : Logic
  Logical Operator2 : Logic
  Logical Operator6 : Logic
  Tilt expired? : lib_CATutils_Timer_Countdown/Timer Countdown  initTime=toa_pfw_time_limit  maxTime=400  timingInput=True  expiredOutput=True  initState=False
  Valve cmd recently became zero : Outport
  wires:
  "Lift cmd, bool"/1 -> Logical Operator/1
  Logical Operator2/1 -> Logical Operator6/2
  Tilt expired?/1 -> Logical Operator4/1  "toa_tilt_timer_expired"
  Logical Operator/1 -> Logical Operator1/1, Lift expired?/1
  Logical Operator6/1 -> Valve cmd recently became zero/1
  Lift expired?/1 -> Logical Operator3/1
  Logical Operator1/1 -> Logical Operator6/1
  Logical Operator3/1 -> Logical Operator1/2
  Logical Operator4/1 -> Logical Operator2/2  "toa_tilt_timer_not_expired"
  "Tilt cmd, bool"/1 -> Logical Operator5/1
  Logical Operator5/1 -> Tilt expired?/1, Logical Operator2/1  "toa_is_not_tilt_valve_cmd"

== matlab function Tip-Off Assist Support Lib/EEF IMU to NEEF gravity vector/Rotation Matrix About Z ==
  data: angle input double; rotMatrix output double
function rotMatrix = fcn(angle)
% Calculates a rotation matrix from an angle in deg
if angle == 0
    rotMatrix = single(eye(3));
    return
end

angleRad = angle / 180.0 * pi;

% Form rotation matrix
a = cos(angleRad);
b = sin(angleRad);
rotMatrix = [
    a, -b, 0;
    b, a, 0;
    0, 0, 1
    ];

== matlab function Tip-Off Assist Support Lib/CPM Payload Send/MATLAB Function ==
  data: pfwStatus input double; pfwPayload input double; pfwIsPrecise input double; outPayload output double; liveStatus input double; livePayload input double; outStatus output double
function [outPayload, outStatus]= sendCpmStatus(pfwStatus, pfwPayload, pfwIsPrecise, liveStatus, livePayload)

if pfwIsPrecise && (pfwStatus == TipAssistSecPfwStatus_t.VALID_MEASURING || pfwStatus == TipAssistSecPfwStatus_t.VALID_NOT_MEASURING)
	outStatus = TipAssistSendCpmStatus_t.PSEUDO_FRICTIONLESS;
    outPayload = pfwPayload;
elseif liveStatus == TipAssistLiveWeighStatus_t.VALID
    outStatus = TipAssistSendCpmStatus_t.LIVE;
    outPayload = livePayload;
else
    outStatus = TipAssistSendCpmStatus_t.INVALID;
    outPayload = single(NaN);
end

== matlab function Tip-Off Assist Support Lib/Tip-Off Assist Payload/Pseudo-Frictionless Weigh/Weighing Statistics, Secure Latched/One Sided Confidence Limit ==
  data: confidence input double; bound output double; stdev input double
function bound = oneSidedConfBound(confidence, stdev)
% Calculates the size of a confidence interval in terms of half its width.
%
% Inputs:
%   confidence
%   Confidence that the resulting bound will enclose the true value.
%
%   stdev
%   The observed standard deviation, expressed in the same units as
%   bound. Can be thought of as defining the scale of the normal
%   distribution that we are assuming represents the data we are sampling.
%
%   Potential units for the arguments are percent of rated payload or
%   payload.
%
% Outputs:
%   bound
%   Bound of the confidence interval, expressed in the same units as stdev.
%   
%   For lower bound, the true value will lie above the mean minus this
%   value.
%   The opposite is true for an upper bound.
%   
% Inspired from pcs_calculate_confidence() in pcs_io.c

% Table of confidence vs one-sided confidence interval bound.
% Units of confidence decimal percent and the ratio of standard
% deviation of a standard normal distribution.
xConfidenceOneSided = [0.500000000000000,0.617911422000000,0.691462461000000,0.758036347000000,0.815939873500000,0.864333838000000,0.903199463500000,0.933192771500000,0.955434528500000,0.971283436000000,0.982135576500000,0.989275889000000,0.993790334000000,0.996533026000000,0.998650102000000,0.999767371000000,1];
yStdevRatio = [ 0.0, 0.3, 0.5, 0.7, 0.9, 1.1, 1.3, 1.5, 1.7, 1.9, 2.1, 2.3, 2.5, 2.7, 3.0, 3.5, 4.0 ];
stdev_ratio = interp1(xConfidenceOneSided, yStdevRatio, confidence);
bound = stdev_ratio * stdev;

== matlab function Tip-Off Assist Support Lib/Tip-Off Assist Payload/Pseudo-Frictionless Weigh/Weighing Statistics, Secure Latched/Two Sided Confidence Limit ==
  data: confidence input double; bound output double; stdev input double
function bound = TwoSidedConfBound(confidence, stdev)
% Calculates the size of a confidence interval in terms of half its width.
%
% Inputs:
%   confidence
%   Confidence that the resulting bound will enclose the true value.
%
%   stdev
%   The observed standard deviation, expressed in the same units as
%   bound. Can be thought of as defining the scale of the normal
%   distribution that we are assuming represents the data we are sampling.
%
%   Potential units for the arguments are percent of rated payload or
%   payload.
%
% Outputs:
%   bound
%   Bound of the confidence interval, expressed in the same units as stdev.
%   
%   For lower bound, the true value will lie above the mean minus this
%   value.
%   The opposite is true for an upper bound.
%   
% Inspired from pcs_calculate_confidence() in pcs_io.c

% Table of confidence vs two-sided confidence interval bound.
% Units of confidence decimal percent and the ratio of standard
% deviation of a standard normal distribution.
xConfidenceTwoSided = [ 0.0, 0.235822844, 0.382924922, 0.516072694, 0.631879747, 0.728667676, 0.806398927, 0.866385543, 0.910869057, 0.942566872, 0.964271153, 0.978551778, 0.987580668, 0.993066052, 0.997300204, 0.999534742, 1.0 ];
yStdevRatio = [ 0.0, 0.3, 0.5, 0.7, 0.9, 1.1, 1.3, 1.5, 1.7, 1.9, 2.1, 2.3, 2.5, 2.7, 3.0, 3.5, 4.0 ];
stdev_ratio = interp1(xConfidenceTwoSided, yStdevRatio, confidence);
bound = stdev_ratio * stdev;

== matlab function Tip-Off Assist Support Lib/Tip-Off Assist Payload/Pseudo-Frictionless Weigh/Statistics Estimation1/MATLAB Function ==
  data: newSample input double; meanEst output double; stdevEst output double; filterFactor input double; reset input double; resetSample input double; resetVariance input double
function [meanEst, stdevEst] = fcn(newSample, filterFactor, reset, resetSample, resetVariance)
% Implements a running mean and standard deviation estimate.
% Formula from:
%   Estimation of Variance by a Recursive Equation
%   by M. Melvin Bruce, October 1969, Langley Research Center (NASA)
% Adapted from PCS's pcs_io.c file.

persistent lastMeanEst lastVarianceEst;

% Init to a high variance to ensure confidence is initially low.
% Init to a high mean so the true value is always approached from above,
% which will ensure a non-warmed-up filter errs high, which will cause
% Tip-Off Assist to err low to prevent truck overload.
if isempty(lastMeanEst) || reset
    lastMeanEst = single(resetSample);
    lastVarianceEst = single(resetVariance);
end

A = 1 - filterFactor;   % "A" from the NASA paper
meanEst = A * lastMeanEst + (1.0 - A) * newSample;
varianceEst = A * lastVarianceEst + (1.0 - A) * (1.0 + A) * (newSample - lastMeanEst) * (newSample - lastMeanEst) / 2.0;
stdevEst = sqrt(varianceEst);

% For next time...
lastMeanEst = meanEst;
lastVarianceEst = varianceEst;
end

== matlab function Tip-Off Assist Support Lib/Tip-Off Assist Payload/Pseudo-Frictionless Weigh/Secure Payload Status ==
  data: inputsBad input double; latched input double; status output double; measCondOk input double; secureAssumed input double
function status = securePfwStatus(inputsBad, latched, measCondOk, secureAssumed)

if inputsBad
    status = TipAssistSecPfwStatus_t.FAULT;
elseif latched && measCondOk && secureAssumed
    % Let consumers know that PFW is valid and may improve in confidence
    status = TipAssistSecPfwStatus_t.VALID_MEASURING;
elseif latched && ~measCondOk && secureAssumed
    % Let consumers know that PFW is valid, but won't improve in confidence
    status = TipAssistSecPfwStatus_t.VALID_NOT_MEASURING;
elseif ~latched && measCondOk && secureAssumed
    % Let consumers know that PFW is likely about to become valid
    status = TipAssistSecPfwStatus_t.PENDING;
else
    status = TipAssistSecPfwStatus_t.INVALID;
end
